simulink model "simulink_scheme_task31"  (R2023b)
settings: Solver=ode4  StartTime=0.0  StopTime=simulationParameters.T_sim  FixedStep=simulationParameters.T_integration  RelTol=1e-3
values from neighbouring files (symbols this model uses):
  nInput = size(B,2)    [buildCondMatrices.m]    (also in main_task31.m; main_task32.m; main_task33.m)
  predictedHorizon = 100    [main_task31.m]    (also in main_task32.m; main_task33.m)
  predictionData = buildCondMatrices(A,B,C,Q,R,F,f,predictedHorizon)    [main_task31.m]    (also in main_task32.m; main_task33.m)
  simulationParameters = loadSimulationParameter    [main_task31.m]    (also in main_task32.m; main_task33.m)
undefined symbols (not defined in the file or in its folder): linearModel, MPCcontroller
settings Model: Creator=william  LastModifiedBy=william
settings DataIOCC: ReturnWorkspaceOutputs=off
settings ConfigComp: CovBoundaryAbsTol=1.0e-5

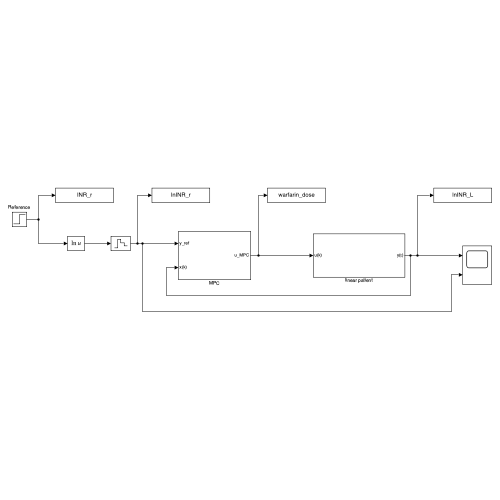
[thumbnail: Simulink's stored preview of the top-level diagram]
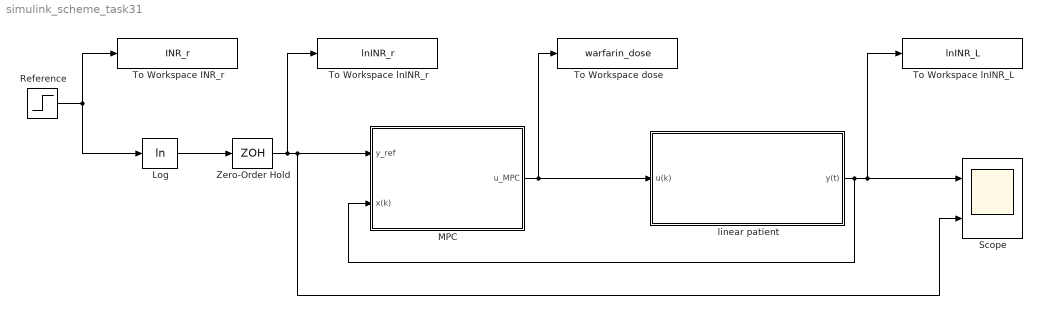
== system simulink_scheme_task31 ==
  Log : Math  Operator=log
  MPC : Subsystem
  Reference : Step  Time=2*24  Before=1  After=2.5  SampleTime=simulationParameters.Ts
  Scope : Scope  NumInputPorts=2
  To Workspace INR_r : ToWorkspace  VariableName=INR_r  SaveFormat=Structure With Time  SampleTime=-1
  To Workspace dose : ToWorkspace  VariableName=warfarin_dose  SaveFormat=Structure With Time  SampleTime=-1
  To Workspace lnINR_L : ToWorkspace  VariableName=lnINR_L  SaveFormat=Structure With Time  SampleTime=-1
  To Workspace lnINR_r : ToWorkspace  VariableName=lnINR_r  SaveFormat=Structure With Time  SampleTime=-1
  Zero-Order Hold : ZeroOrderHold  SampleTime=simulationParameters.Ts
  linear patient : Subsystem
  wires:
  Reference/1 -> Log/1, To Workspace INR_r/1
  Log/1 -> Zero-Order Hold/1
  Zero-Order Hold/1 -> Scope/2, MPC/1(y_ref), To Workspace lnINR_r/1
  MPC/1(u_MPC) -> To Workspace dose/1, linear patient/1(u(k))
  linear patient/1(y(t)) -> To Workspace lnINR_L/1, Scope/1, MPC/2(x(k))

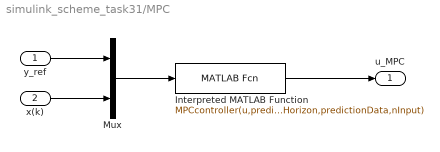
== system simulink_scheme_task31/MPC ==
  y_ref : Inport
  x(k) : Inport  Port=2
  Interpreted MATLAB Function : MATLABFcn  MATLABFcn=MPCcontroller(u,predictedHorizon,predictionData,nInput)
  Mux : Mux  Inputs=2
  u_MPC : Outport
  wires:
  y_ref/1 -> Mux/1
  x(k)/1 -> Mux/2
  Mux/1 -> Interpreted MATLAB Function/1
  Interpreted MATLAB Function/1 -> u_MPC/1

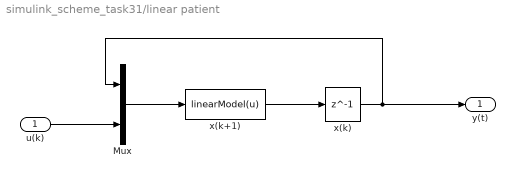
== system simulink_scheme_task31/linear patient ==
  u(k) : Inport
  Mux : Mux  Inputs=2
  x(k) : Delay  DelayLength=1
  x(k+1) : MATLABFcn  MATLABFcn=linearModel(u)  OutputDimensions=1
  y(t) : Outport
  wires:
  x(k)/1 -> y(t)/1, Mux/1
  u(k)/1 -> Mux/2
  Mux/1 -> x(k+1)/1
  x(k+1)/1 -> x(k)/1
